simulink model "DesktopRobotSimuModel"  (R2026b)
settings: Solver=FixedStepDiscrete  StopTime=inf  FixedStep=0.01  EnableMultiTasking=on
PostLoadFcn:
  | robotRoot = fileparts(fileparts(get_param(bdroot,'FileName'))); addpath(fullfile(robotRoot,'scripts'), fullfile(robotRoot,'blocks','oled','Oled_eyes'), fullfile(robotRoot,'blocks','buzzer','Buzzer_tone'));
InitFcn:
  | robotRoot = fileparts(fileparts(get_param(bdroot,'FileName'))); addpath(fullfile(robotRoot,'scripts'), fullfile(robotRoot,'blocks','oled','Oled_eyes'), fullfile(robotRoot,'blocks','buzzer','Buzzer_tone'));
  | params
undefined symbols (not defined in the file): adcMax, alignLeft, alignRight, backTime, backward, brake, dance, dancePeriod, dirLeft, dirRight, endHappy, faceCurious, faceHappy, faceNeutral, faceSad, faceSleep, faceSurprised, highVolt, lowBattDelay, lowVolt, petOn, pwmMax, pwmMin, rampTime, sideBoth, sideLeft, sideRight, sleepTime, sndHappy, sndLowBatt, sndNone, sndOops, sndSleep, sndWake, soundOn, speedAlign, speedBack, speedDance, speedTurn, speedWander, stopTime, tauBatt, Ts, turnTime, voidValue, vRef, wander, wanderGo, wanderPause, wanderTurn, wanderTurnProb, wanderWait
libraries: arduinolib x8, simulink x1
settings Model: SILPILModeSetting=veronly  Creator=cyril  LastModifiedBy=cyril
settings SolverCC: AutoInsertRateTranBlk=on
settings OptimizationCC: DifferentSizesBufferReuse=on  EnhancedBackFolding=on  MaxStackSize=64  OptimizationCustomize=off  OptimizeBlockOrder=speed
settings DebuggingCC: ParameterTunabilityLossMsg=error
settings HardwareCC: ProdHWDeviceType=ARM Compatible->ARM Cortex  ProdLargestAtomicFloat=Double  ProdLargestAtomicInteger=Long  UseEmbeddedCoderFeatures=off  UseSimulinkCoderFeatures=off
settings SFSimCC: MATLABDynamicMemAlloc=off
settings RTWCC: BuildConfiguration=Faster Runs  Description=Embedded Coder  HardwareBoard=Arduino Nano R4  SystemTargetFile=ert.tlc  TLCOptions=-aInlineSetEventsForThisBaseRateFcn=TLC_FALSE -aSuppressMultiTaskScheduler=TLC_FALSE -aRateBasedStepFcn=1  TemplateMakefile=ert_default_tmf  Toolchain=Arduino ARM M4
settings CodeAppCC: ForceParamTrailComments=on  OperatorAnnotations=on
settings ERTTargetCC: CombineSignalStateStructs=on  ERTCustomFileBanners=off  ExtModeAutomaticAllocSize=off  ExtModeIntrfLevel=Level2 - Open  ExtModeMexFile=ext_xcp  ExtModeStaticAlloc=on  ModelStepFunctionPrototypeControlCompliant=off  SupportContinuousTime=on  SupportNonInlinedSFcns=on  SupportVariableSizeSignals=on

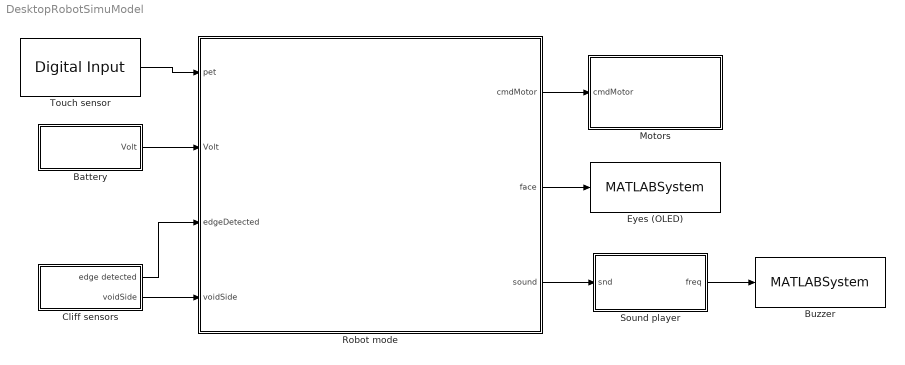
== system DesktopRobotSimuModel ==
  Battery : Subsystem
  Buzzer : MATLABSystem  System=Buzzer_tone  Pin=int8(3)
      mask Type: Buzzer_tone
  Cliff sensors : Subsystem
  Eyes (OLED) : MATLABSystem  System=Oled_eyes  BlockParameter=int8(0)
      mask Type: Oled_eyes
  Motors : Subsystem
  Robot mode : Stateflow chart  TreatAsAtomicUnit=on
  Sound player : MATLAB Function  TreatAsAtomicUnit=on
  Touch sensor : arduinolib/Digital Input  pinNumber=11  mode=Default  Direction=input  SampleTime=-1  blockPlatform=arduino
  wires:
  Touch sensor/1 -> Robot mode/1(pet)
  Battery/1(Volt) -> Robot mode/2(Volt)
  Cliff sensors/1(edge detected) -> Robot mode/3(edgeDetected)
  Cliff sensors/2(voidSide) -> Robot mode/4(voidSide)
  Robot mode/3(sound) -> Sound player/1(snd)
  Robot mode/2(face) -> Eyes (OLED)/1
  Robot mode/1(cmdMotor) -> Motors/1(cmdMotor)
  Sound player/1(freq) -> Buzzer/1

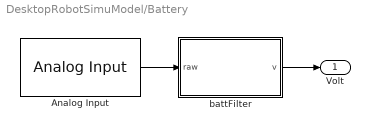
== system DesktopRobotSimuModel/Battery ==
  Analog Input : arduinolib/Analog Input  pinNumber=0  ReadResultsOnly=off  ConversionTriggerSource=Software  ExternalTriggerType=uint32( 0 )  OutputDataType=uint16  EnableConversionCompleteNotify=off  EnableOuputStatus=off  SampleTime=Ts  blockPlatform=arduino
  battFilter : MATLAB Function  TreatAsAtomicUnit=on
  Volt : Outport
  wires:
  battFilter/1(v) -> Volt/1
  Analog Input/1 -> battFilter/1(raw)

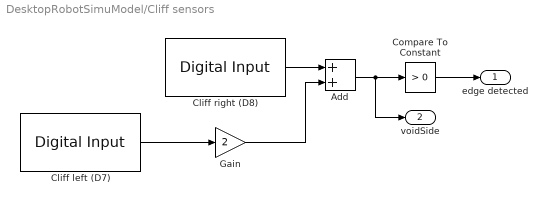
== system DesktopRobotSimuModel/Cliff sensors ==
  Add : Sum
  Cliff left (D7) : arduinolib/Digital Input  pinNumber=7  mode=Default  Direction=input  SampleTime=-1  blockPlatform=arduino
  Cliff right (D8) : arduinolib/Digital Input  pinNumber=8  mode=Default  Direction=input  SampleTime=-1  blockPlatform=arduino
  Compare To Constant : simulink/Logic and Bit Operations/Compare To Constant  relop=>  const=0  OutDataTypeStr=boolean
  Gain : Gain  Gain=2
  edge detected : Outport
  voidSide : Outport  Port=2
  wires:
  Compare To Constant/1 -> edge detected/1
  Add/1 -> voidSide/1, Compare To Constant/1
  Cliff right (D8)/1 -> Add/1
  Cliff left (D7)/1 -> Gain/1
  Gain/1 -> Add/2

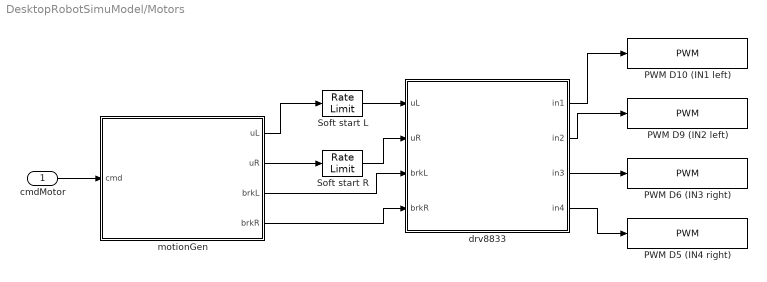
== system DesktopRobotSimuModel/Motors ==
  cmdMotor : Inport
  PWM D10 (IN1 left) : arduinolib/PWM  pinNumber=10  frequencyType=Default  desiredFrequency=490.2  achievableFrequency=490.2
  PWM D5 (IN4 right) : arduinolib/PWM  pinNumber=5  frequencyType=Default  desiredFrequency=490.2  achievableFrequency=490.2
  PWM D6 (IN3 right) : arduinolib/PWM  pinNumber=6  frequencyType=Default  desiredFrequency=490.2  achievableFrequency=490.2
  PWM D9 (IN2 left) : arduinolib/PWM  pinNumber=9  frequencyType=Default  desiredFrequency=490.2  achievableFrequency=490.2
  Soft start L : RateLimiter  RisingSlewLimit=1/rampTime  FallingSlewLimit=-1/rampTime  SampleTimeMode=inherited
  Soft start R : RateLimiter  RisingSlewLimit=1/rampTime  FallingSlewLimit=-1/rampTime  SampleTimeMode=inherited
  drv8833 : MATLAB Function  TreatAsAtomicUnit=on
  motionGen : MATLAB Function  TreatAsAtomicUnit=on
  wires:
  cmdMotor/1 -> motionGen/1(cmd)
  motionGen/3(brkL) -> drv8833/3(brkL)
  motionGen/2(uR) -> Soft start R/1
  motionGen/1(uL) -> Soft start L/1
  motionGen/4(brkR) -> drv8833/4(brkR)
  drv8833/1(in1) -> PWM D10 (IN1 left)/1
  Soft start R/1 -> drv8833/2(uR)
  Soft start L/1 -> drv8833/1(uL)
  drv8833/2(in2) -> PWM D9 (IN2 left)/1
  drv8833/3(in3) -> PWM D6 (IN3 right)/1
  drv8833/4(in4) -> PWM D5 (IN4 right)/1

== matlab function DesktopRobotSimuModel/Motors/motionGen ==
  data: cmd input; uL output; uR output; brkL output; brkR output; Ts parameter; wander parameter; dance parameter; backward parameter; alignRight parameter; alignLeft parameter; speedWander parameter; speedTurn parameter; speedDance parameter; speedBack parameter; speedAlign parameter; wanderGo parameter; wanderTurn parameter; wanderPause parameter; wanderTurnProb parameter; dancePeriod parameter
function [uL, uR, brkL, brkR] = motionGen(cmd, Ts, wander, dance, backward, alignRight, alignLeft, speedWander, speedTurn, speedDance, speedBack, speedAlign, wanderGo, wanderTurn, wanderPause, wanderTurnProb, dancePeriod)
% MOTION GENERATOR - turns the chart's motor command (cmdMotor) into a
% target speed for each wheel (-1..1, + = forward) and a brake flag per wheel.
% Parameters come from params.m (command codes, speeds, wander/dance timing, Ts).
persistent lastCmd t tc phase dur turnDir seed
if isempty(lastCmd)
    lastCmd = -1; t = 0; tc = 0; phase = 0; dur = 1; turnDir = 1; seed = 20261101;
end
if cmd ~= lastCmd               % new command: restart its little sequence
    t = 0; tc = 0; phase = 0; dur = wanderPause(1);
    lastCmd = cmd;
end
t = t + Ts;
tc = tc + Ts;                   % time since the command changed

uL = 0; uR = 0; brkL = false; brkR = false;
if tc < 0.2 && cmd ~= 0         % short coast between two moves: the wheels slow
    return                      % down before the next one (no current spike)
end

if cmd == wander
    % random sequence: pause -> (short step forward OR small turn) -> pause ...
    % Both wheels always turn forward: no spinning on the spot, no reversing
    % (there is no cliff sensor at the back).
    if t >= dur
        t = 0;
        [r1, seed] = rnd(seed);
        [r2, seed] = rnd(seed);
        if phase ~= 0                       % a move just ended -> pause
            phase = 0;
            dur = wanderPause(1) + r1*(wanderPause(2) - wanderPause(1));
        elseif r1 < wanderTurnProb          % small turn, random side
            phase = 2;
            if r2 < 0.5, turnDir = 1; else, turnDir = -1; end
            [r3, seed] = rnd(seed);
            dur = wanderTurn(1) + r3*(wanderTurn(2) - wanderTurn(1));
        else                                % small step forward
            phase = 1;
            dur = wanderGo(1) + r2*(wanderGo(2) - wanderGo(1));
        end
    end
    if phase == 1
        uL = speedWander;        uR = speedWander;
    elseif phase == 2
        % turn: one wheel forward, the other one stopped (never backwards)
        if turnDir > 0
            uL = speedTurn;      uR = 0;                 % turn to the right
        else
            uL = 0;              uR = speedTurn;         % turn to the left
        end
    else
        brkL = true;             brkR = true;
    end

elseif cmd == dance
    % gentle wiggle: one wheel at a time, with a short gap before each
    % change of direction (both motors reversing at once reset the Nano)
    k = mod(t, dancePeriod) / dancePeriod;   % position in one wiggle, 0..1
    if k < 0.2
        uL = speedDance;                     % left wheel forward
    elseif k >= 0.25 && k < 0.45
        uL = -speedDance;                    % left wheel back
    elseif k >= 0.5 && k < 0.7
        uR = speedDance;                     % right wheel forward
    elseif k >= 0.75 && k < 0.95
        uR = -speedDance;                    % right wheel back
    end                                      % gaps: wheels slow down to 0 (soft start)

elseif cmd == backward
    uL = -speedBack; uR = -speedBack;

elseif cmd == alignRight            % right wheel braked, left wheel slowly forward
    uL = speedAlign; brkR = true;

elseif cmd == alignLeft             % left wheel braked, right wheel slowly forward
    uR = speedAlign; brkL = true;

else                                % brake (and any unknown code)
    brkL = true; brkR = true;
end
end

function [r, s] = rnd(s)
% Park-Miller pseudo-random number in (0,1)
s = mod(s*16807, 2147483647);
r = s/2147483647;
end

== matlab function DesktopRobotSimuModel/Battery/battFilter ==
  data: raw input; v output; vRef parameter; adcMax parameter; Ts parameter; tauBatt parameter
function v = battFilter(raw, vRef, adcMax, Ts, tauBatt)
% BATTERY VOLTAGE - raw ADC count on A0 -> battery voltage [V], smoothed by a
% first-order low-pass (time constant tauBatt) so that motor start-up dips
% do not send the robot to Deep_Sleep. Starts directly at the first reading.
persistent y
vin = double(raw)*vRef/adcMax;
if isempty(y), y = vin; end
y = y + (Ts/tauBatt)*(vin - y);
v = y;
end

== stateflow chart DesktopRobotSimuModel/Robot mode ==
  state Normal
    state NormalBatt
      state Sleep
        entry:
        cmdMotor = brake
        face = faceSleep
        sound = sndSleep
      state Awake
        entry:
        cmdMotor = brake;
        face = faceNeutral
        sound =sndWake
      state Moving
        state Wander
          entry:
          cmdMotor = wander
          face = faceCurious
          sound = sndNone
        state Happy
          entry:
          cmdMotor = dance
          face = faceHappy
          sound = sndHappy
        Wander -> Happy [order 2] : [hasChangedTo(pet, petOn)]
      (default) -> Sleep
      Wander -> Sleep [order 1] : after(sleepTime, sec)
      Sleep -> Awake : [pet == petOn]
      Happy -> Awake : after(endHappy, sec)
      Awake -> Wander [order 2] : after(wanderWait, sec)
      Awake -> Happy [order 1] : [hasChangedTo(pet, petOn)]
    state LowBatt
      state Deep_Sleep
        entry:
        cmdMotor = brake
        face = faceSad
        sound = sndLowBatt
      (default) -> Deep_Sleep
    (default) -> NormalBatt
    NormalBatt -> LowBatt : [duration(Volt <= lowVolt, sec) > lowBattDelay]
    LowBatt -> NormalBatt : [Volt >= highVolt]
  state Edge
    state Wait
      entry:
      cmdMotor = brake
    state Turn_Left
      entry:
      cmdMotor = alignLeft
      face = faceSurprised
      sound = sndNone
    state Stop
      entry:
      cmdMotor = brake
      face = faceSurprised
      sound = sndOops
    state Turn_Right
      entry:
      cmdMotor = alignRight
      face = faceSurprised
      sound = sndNone
    state Backward
      entry:
      cmdMotor = backward
      face = faceSurprised
      sound = sndNone
    (default) -> Stop
    Turn_Left -> Wait : after(turnTime, sec)
    (junction 79) -> Turn_Left [order 1] : [edgeSide == sideRight || edgeSide == sideBoth]
    Turn_Right -> Wait : after(turnTime, sec)
    (junction 79) -> Wait [order 3]
    Stop -> Backward : after(stopTime, sec)
    Backward -> (junction 79) : after(backTime, sec)
    (junction 79) -> Turn_Right [order 2] : [edgeSide == sideLeft]
  (default) -> Normal
  Wait -> Wander
  Moving -> Edge : [edgeDetected == voidValue] {edgeSide = voidSide}
  data: cmdMotor output; petOn parameter; pet input; endHappy parameter; sleepTime parameter; Volt input; lowVolt parameter; highVolt parameter; edgeDetected input; brake parameter; dance parameter; wander parameter; backward parameter; edgeSide local; voidSide input; voidValue parameter; lowBattDelay parameter; stopTime parameter; sideRight parameter; sideLeft parameter; wanderWait parameter; alignLeft parameter; alignRight parameter; sideBoth parameter; face output; faceSleep parameter; sound output; sndNone parameter; faceHappy parameter; faceNeutral parameter; sndHappy parameter; sndWake parameter; faceCurious parameter; faceSurprised parameter; faceSad parameter; sndOops parameter; sndLowBatt parameter; backTime parameter; sndSleep parameter; turnTime parameter

== matlab function DesktopRobotSimuModel/Motors/drv8833 ==
  data: uL input; in1 output; uR input; brkL input; brkR input; in2 output; in3 output; in4 output; dirLeft parameter; dirRight parameter; pwmMin parameter; pwmMax parameter
function [in1, in2, in3, in4] = drv8833(uL, uR, brkL, brkR, dirLeft, dirRight, pwmMin, pwmMax)
% DRV8833 DRIVER - per motor: forward = (PWM, 0), reverse = (0, PWM),
% brake = (255, 255), coast = (0, 0). Duty 0..255 for the Arduino PWM blocks.
% The brake bypasses the soft-start ramp: it acts immediately.
[in1, in2] = bridge(dirLeft*uL,  brkL, pwmMin, pwmMax);
[in3, in4] = bridge(dirRight*uR, brkR, pwmMin, pwmMax);
end

function [a, b] = bridge(u, brk, pMin, pMax)
a = uint8(0); b = uint8(0);
if brk
    a = uint8(255); b = uint8(255);
elseif abs(u) > 0.02
    duty = uint8(round(255*(pMin + (pMax - pMin)*min(abs(u), 1))));
    if u > 0
        a = duty;
    else
        b = duty;
    end
end
end

== matlab function DesktopRobotSimuModel/Sound player ==
  data: snd input; freq output; Ts parameter; soundOn parameter
function freq = soundPlayer(snd, Ts, soundOn)
% SOUND PLAYER - plays a short melody each time the chart asks for a new
% sound code (1 wake, 2 happy, 3 oops, 4 sleep, 5 low battery).
% Output: note frequency in Hz for the Buzzer_tone block (0 = silence).
% F = notes [Hz] (0 = short silence between notes), D = durations [ms].
F = [1047    0 1319    0 1568    0;    % 1 wake     : rising C-E-G
     1568 2093 1568 2093    0 2637;    % 2 happy    : chirpy trill
     1760 1319  880    0    0    0;    % 3 oops     : falling "oh-oh"
      784    0  659    0  523    0;    % 4 sleep    : slow yawn
      440    0  349    0  262    0];   % 5 low batt : sad and low
D = [  70   20   70   20  140    0;
       60   60   60   60   30  160;
       90   90  220    0    0    0;
      160   40  160   40  320    0;
      250   80  250   80  450    0];
N = [5 6 3 5 5];                        % number of notes per melody

persistent lastSnd mel idx tLeft
if isempty(lastSnd)
    lastSnd = 0; mel = 1; idx = 0; tLeft = 0;
end
if snd ~= lastSnd && snd >= 1 && snd <= 5      % new sound requested
    mel = round(snd); idx = 1; tLeft = D(mel, 1);
end
lastSnd = snd;

freq = 0;
if idx > 0
    freq = F(mel, idx) * 0.5;                  % one octave lower: softer, quieter
    tLeft = tLeft - Ts*1000;
    if tLeft <= 0                               % next note
        idx = idx + 1;
        if idx > N(mel)
            idx = 0;                            % melody finished
        else
            tLeft = tLeft + D(mel, idx);
        end
    end
end
if soundOn == 0
    freq = 0;
end
end
